simulink model "bloc"  (R2024a)
settings: Solver=ode4  StartTime=0.0  StopTime=200  FixedStep=0.01  RelTol=1e-3
libraries: fuzblock x1, SignalEditorBlockLib x1
settings Model: Creator=lenov  LastModifiedBy=scide
settings DebuggingCC: UnconnectedInputMsg=warning  UnconnectedOutputMsg=warning  UnconnectedLineMsg=warning
settings ModelReferenceCC: EnableRefExpFcnMdlSchedulingChecks=on
settings RTWCC: GPUComputeCapability=3.5  DLArmComputeVersion=19.05

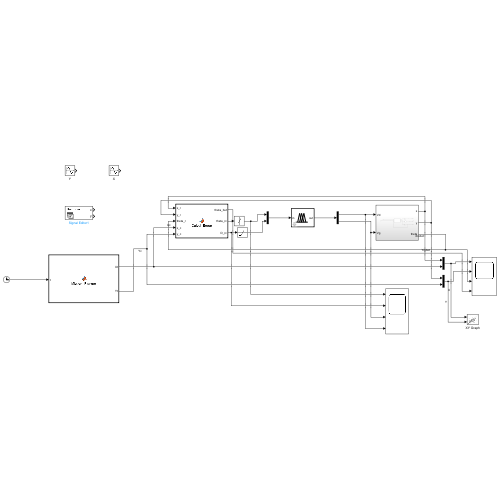
[thumbnail: Simulink's stored preview of the top-level diagram]
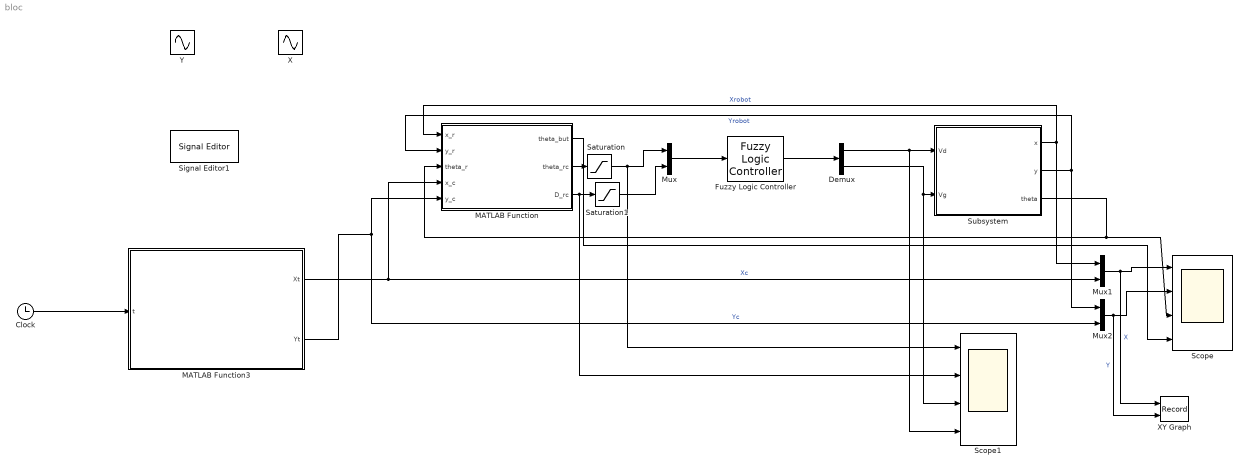
== system bloc ==
  Clock : Clock
  Demux : Demux  Outputs=2
  Fuzzy Logic Controller : fuzblock/Fuzzy Logic  Controller  FIS='RobotStable11.fis'  OutputSampleNumber=101  DataType=double  FuzzifiedInputs=off  RuleFiringStrengths=off  RuleOutputs=off  AggregatedOutputs=off  SimulateUsing=Interpreted execution  OutOfRangeInputValueMessage=warning  NoRuleFiredMessage=warning  EmptyOutputFuzzySetMessage=warning
  MATLAB Function : MATLAB Function  TreatAsAtomicUnit=on
  MATLAB Function3 : MATLAB Function  TreatAsAtomicUnit=on
  Mux : Mux  Inputs=2
  Mux1 : Mux  Inputs=2
  Mux2 : Mux  Inputs=2
  Saturation : Saturate  UpperLimit=pi  LowerLimit=-pi
  Saturation1 : Saturate  UpperLimit=10  LowerLimit=0
  Scope : Scope  NumInputPorts=4
  Scope1 : Scope  NumInputPorts=4
  Signal Editor1 : SignalEditorBlockLib/Signal Editor  FileName=C:\GSEA_Génie_des_Systèmes_Electronique_et_Automatiques\Robotique\Robotique_2CI\Matlab_TP_Robotique\TpModelisation\Robot Manipulateur 2DOF\signal.mat  ActiveScenario=Scenario  ActiveSignal=y  IsBus=off  OutputBusObjectStr=Bus: BusObject  SampleTime=0  ZeroCross=off  OutputAfterFinalValue=Setting to zero  Unit=inherit  PreserveSignalName=on  ApplySigPropsToAllScenarios=on  ApplySigPropsToAllSignals=on
  Subsystem : Subsystem
  X : Sin  Amplitude=5  Frequency=0.1  SampleTime=0
  XY Graph : Record  FileSettingsInternal="{\"entries\":[{\"content\":{\"excelSettings\":{\"content\":{},\"type\":\"Streamout.ExcelSettings\"}},\"type\":\"Streamout.FileSettingStorage\",\"uuid\":\"\"}],\"packageUris\":[\"http:\\/\\/schema.mathworks.com\\/mf0\\/streamout_blocks\\/R2020a\"],\"version\":\"1.0\"}"  Layout=[1 1]  SignalsInternal="{\"entries\":[{\"content\":{\"signals\":[{\"content\":{\"blockPath\":[],\"dimensions\":[2],\"domain\":\"\",\"hasChildren\":true,\"lineColor\":\"#a2142f\",\"lineWidth\":2,\"port\":1,\"sid\":[\"\"],\"signalID\":1,\"signalName\":\"X\"},\"type\":\"RecordBlkView.Signal\",\"uuid\":\"\"},{\"content\":{\"blockPath\":[],\"channel\":[1],\"dimensions\":[2],\"domain\":\"\",\"lineColor\":\"#ff13a6\",\"lineWidth\":2,\"parentID\":1,\"plots\":[ 1 ],\"port\":1,\"sid\":[\"\"],\"signalID\":2,\"signalName\":\"X\"},\"type\":\"RecordBlkView.Signal\",\"uuid\":\"\"},{\"content\":{\"blockPath\":[],\"dimensions\":[2],\"domain\":\"\",\"hasChildren\":true,\"lineColor\":\"#ff6929\",\"lineWidth\":2,\"port\":2,\"sid\":[\"\"],\"signalID\":3,\"signalName\":\"Y\"},\"type\":\"RecordBlkView.Signal\",\"uuid\":\"\"},{\"content\":{\"blockPath\":[],\"channel\":[1],\"dimensions\":[2],\"domain\":\"\",\"lineColor\":\"#22b573\",\"lineWidth\":2,\"parentID\":3,\"plots\":[ 1 ],\"port\":2,\"sid\":[\"\"],\"signalID\":4,\"signalName\":\"Y\"},\"type\":\"RecordBlkView.Signal\",\"uuid\":\"\"},{\"content\":{\"blockPath\":[],\"channel\":[2],\"dimensions\":[2],\"domain\":\"\",\"lineColor\":\"#0072bd\",\"lineWidth\":2,\"parentID\":1,\"plots\":[ 1 ],\"port\":1,\"sid\":[\"\"],\"signalID\":5,\"signalName\":\"X\"},\"type\":\"RecordBlkView.Signal\",\"uuid\":\"\"},{\"content\":{\"blockPath\":[],\"channel\":[2],\"dimensions\":[2],\"domain\":\"\",\"lineColor\":\"#d95319\",\"lineWidth\":2,\"parentID\":3,\"plots\":[ 1 ],\"port\":2,\"sid\":[\"\"],\"signalID\":6,\"signalName\":\"Y\"},\"type\":\"RecordBlkView.Signal\",\"uuid\":\"\"}]},\"type\":\"RecordBlkView.InputSignals\",\"uuid\":\"\"}],\"packageUris\":[\"http:\\/\\/schema.mathworks.com\\/mf0\\/streamout_blocks\\/R2020a\"],\"version\":\"1.0\"}"  VisualizationBindings="{\"xyplotplugin\":{\"info\":[{\"series\":[{\"bindingParametersList\":[{\"parameter\":\"X-Axis\",\"signalID\":5,\"signalName\":\"X(2)\"},{\"parameter\":\"Y-Axis\",\"signalID\":6,\"signalName\":\"Y(2)\"}],\"seriesID\":0},{\"bindingParametersList\":[{\"parameter\":\"X-Axis\",\"signalID\":2,\"signalName\":\"X(1)\"},{\"parameter\":\"Y-Axis\",\"signalID\":4,\"signalName\":\"Y(1)\"}],\"seriesID\":1}],\"subplotID\":1}]}}"  CompatibilityTag=XY
  Y : Sin  Amplitude=5  Frequency=0.1  Phase=pi/2  SampleTime=0
  wires:
  Demux/1 -> Scope1/4, Subsystem/1(Vd)
  Demux/2 -> Scope1/3, Subsystem/2(Vg)
  MATLAB Function3/1(Xt) -> MATLAB Function/4(x_c), Mux1/2  "Xc"
  MATLAB Function3/2(Yt) -> MATLAB Function/5(y_c), Mux2/2  "Yc"
  Mux/1 -> Fuzzy Logic Controller/1
  Subsystem/1(x) -> Mux1/1, MATLAB Function/1(x_r)  "Xrobot"
  Subsystem/2(y) -> Mux2/1, MATLAB Function/2(y_r)  "Yrobot"
  Subsystem/3(theta) -> Scope/3, MATLAB Function/3(theta_r)
  Mux1/1 -> XY Graph/1, Scope/1  "X"
  Mux2/1 -> XY Graph/2, Scope/2  "Y"
  Fuzzy Logic Controller/1 -> Demux/1
  MATLAB Function/1(theta_but) -> Scope/4
  MATLAB Function/2(theta_rc) -> Saturation/1
  MATLAB Function/3(D_rc) -> Saturation1/1, Scope1/2
  Saturation/1 -> Scope1/1, Mux/1
  Saturation1/1 -> Mux/2
  Clock/1 -> MATLAB Function3/1(t)

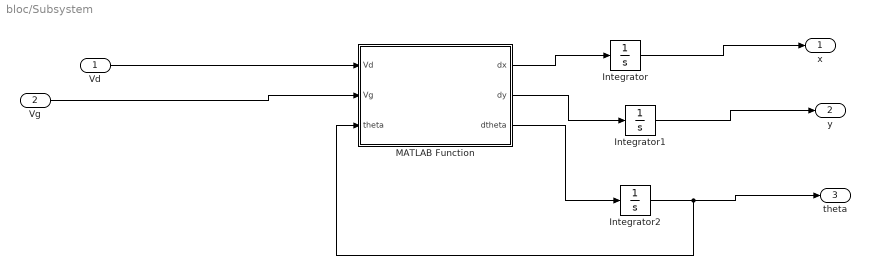
== system bloc/Subsystem ==
  Vd : Inport
  Vg : Inport  Port=2
  Integrator : Integrator
  Integrator1 : Integrator
  Integrator2 : Integrator
  MATLAB Function : MATLAB Function  TreatAsAtomicUnit=on
  x : Outport
  y : Outport  Port=2
  theta : Outport  Port=3
  wires:
  MATLAB Function/3(dtheta) -> Integrator2/1
  MATLAB Function/2(dy) -> Integrator1/1
  Vg/1 -> MATLAB Function/2(Vg)
  Integrator1/1 -> y/1
  Integrator/1 -> x/1
  MATLAB Function/1(dx) -> Integrator/1
  Vd/1 -> MATLAB Function/1(Vd)
  Integrator2/1 -> MATLAB Function/3(theta), theta/1

== matlab function bloc/MATLAB Function ==
  data: theta_but output; theta_rc output; D_rc output; x_r input; y_r input; theta_r input; x_c input; y_c input
function [theta_but, theta_rc, D_rc] = Calcul_Erreur(x_r, y_r, theta_r, x_c, y_c)
    
    
    ex = x_c - x_r;
    ey = y_c - y_r;
   
    dist_sq = ex^2 + ey^2;
    D_rc = sqrt(dist_sq); % Distance réelle
    
   
    seuil_stabilite = 0.05; 
    
    if D_rc < seuil_stabilite
   
        theta_rc = 0;
        theta_but = theta_r;
    else
        
        theta_but = atan2(ey, ex); 

       
        err_brute = theta_but - theta_r;
        
       
        theta_rc = atan2(sin(err_brute), cos(err_brute));
    end
    
end

== matlab function bloc/Subsystem/MATLAB Function ==
  data: Vd input; dx output; Vg input; theta input; dy output; dtheta output
function [dx, dy, dtheta] = Modele_Robot(Vd, Vg, theta)
    L=0.15;
    V = (Vd + Vg) / 2;      
    w = (Vd - Vg) / (2 * L); 

    dx     = V * cos(theta);
    dy     = V * sin(theta);
    dtheta = w;
end

== matlab function bloc/MATLAB Function3 ==
  data: t input; Xt output; Yt output
function [Xt, Yt] = Mission_Planner(t)
    % Configuration de la mission
    T_fin_trajectoire = 63; % Après un tour complet (environ 63s), on va se garer
    
    % Phase 1 : Suivi de trajectoire (Figure en 8)
    if t < T_fin_trajectoire
        % Paramètres du 8 (Lissajous)
        A = 10;
        omega = 0.1;
        
        Xt = A * sin(omega * t);
        Yt = 5 * sin(2 * omega * t);
        
    % Phase 2 : Parking (Retour à la base)
    else
        % Coordonnées de la base de recharge (Parking)
        % On définit une cible fixe.
        Xt = 5;  
        Yt = 5;
    end
end
